simulink model "pgfm_ctrl_analysis"  (R2026b)
settings: Solver=ode23t  StopTime=param.sim.simlength  FixedStep=param.sim.tc  MaxStep=param.glb_time.tc  RelTol=1e-4
values from neighbouring files (symbols this model uses):
  param = add_template_extras(param, options)    [init_model.m]
undefined symbols (not defined in the file or in its folder): magnitude
libraries: fl_lib x99, nesl_utility x59, afe_uvw_ctrl x15, discrete_time_low_pass_filter x3, threephase_inductor_lib x3, dclink_for_two_levels x3, three_phase_pwm_modulator x3, ideal_bridges_lib x3, lithium_ion_battery x1, three_phase_voltage_with_frt_emulator_mfcn x1
(part 3 of 6)

== system pgfm_ctrl_analysis/afe_abc_inv_psm_mod2/afe/three_phase_inverter_ideal_switch_based_model ==
  gate_commands : Inport
  PS Terminator : fl_lib/Physical Signals/Sinks/PS Terminator
  PS Terminator1 : fl_lib/Physical Signals/Sinks/PS Terminator
  Simulink-PS Converter : nesl_utility/Simulink-PS Converter  PhysicalDomain=network_engine_domain  SubClassName=ps_input  LeftPortType=input  RightPortType=output  PseudoPeriodic=off  Frequencies=[]  NoiseDistribution=none  NoiseParameters=[]  Unit=V  AffineConversion=off  FilteringAndDerivatives=provide  SimscapeFilterOrder=1  InputFilterTimeConstant=0.001  UdotUserProvided=0
  Three-Phase Bridge (ideal) : ideal_bridges_lib/Three-Phase Bridge (ideal)  Vth=2.5 V  Ron=1e-3 Ohm  Goff=1e-6 1/Ohm  cap_dc=ideal_bridges.onoff.on  Cdc=2e-3 F  Vdc0=0 V  ind_ac=ideal_bridges.onoff.on  L=1e-3 H  RL=10e-3 Ohm  vdc_specify=off  vdc_priority=None  vdc=0 V  vdc_nominal_specify=off  vdc_nominal_value=1  vdc_nominal_unit=V  ic_specify=off  ic_priority=None  ic=0 A  ic_nominal_specify=off  ic_nominal_value=1  ic_nominal_unit=A  vm_a_specify=off  vm_a_priority=None  vm_a=0 V  vm_a_nominal_specify=off  vm_a_nominal_value=1  vm_a_nominal_unit=V  vm_b_specify=off  vm_b_priority=None  vm_b=0 V  vm_b_nominal_specify=off  vm_b_nominal_value=1  vm_b_nominal_unit=V  vm_c_specify=off  vm_c_priority=None  vm_c=0 V  vm_c_nominal_specify=off  vm_c_nominal_value=1  vm_c_nominal_unit=V  i_ah_specify=off  i_ah_priority=None  i_ah=0 A  i_ah_nominal_specify=off  i_ah_nominal_value=1  i_ah_nominal_unit=A  i_al_specify=off  i_al_priority=None  i_al=0 A  i_al_nominal_specify=off  i_al_nominal_value=1  i_al_nominal_unit=A  i_bh_specify=off  i_bh_priority=None  i_bh=0 A  i_bh_nominal_specify=off  i_bh_nominal_value=1  i_bh_nominal_unit=A  i_bl_specify=off  i_bl_priority=None  i_bl=0 A  i_bl_nominal_specify=off  i_bl_nominal_value=1  i_bl_nominal_unit=A  i_ch_specify=off  i_ch_priority=None  i_ch=0 A  i_ch_nominal_specify=off  i_ch_nominal_value=1  i_ch_nominal_unit=A  i_cl_specify=off  i_cl_priority=None  i_cl=0 A  i_cl_nominal_specify=off  i_cl_nominal_value=1  i_cl_nominal_unit=A  i_a_specify=off  i_a_priority=None  i_a=0 A  i_a_nominal_specify=off  i_a_nominal_value=1  i_a_nominal_unit=A  i_b_specify=off  i_b_priority=None  i_b=0 A  i_b_nominal_specify=off  i_b_nominal_value=1  i_b_nominal_unit=A  i_c_specify=off  i_c_priority=None  i_c=0 A  i_c_nominal_specify=off  i_c_nominal_value=1  i_c_nominal_unit=A
  udc(+) : PMIOPort  Side=Left
  u : PMIOPort  Port=2  Side=Right
  v : PMIOPort  Port=3  Side=Right
  udc(-) : PMIOPort  Port=4  Side=Left
  w : PMIOPort  Port=5  Side=Right
  wires:
  gate_commands/1 -> Simulink-PS Converter/1
  connections:
  PS Terminator1/LConn1 -- Three-Phase Bridge (ideal)/LConn4
  PS Terminator/LConn1 -- Three-Phase Bridge (ideal)/LConn3
  Simulink-PS Converter/RConn1 -- Three-Phase Bridge (ideal)/RConn4
  Three-Phase Bridge (ideal)/RConn1 -- u/RConn1
  Three-Phase Bridge (ideal)/LConn2 -- udc(-)/RConn1
  Three-Phase Bridge (ideal)/RConn2 -- v/RConn1
  Three-Phase Bridge (ideal)/RConn3 -- w/RConn1
  Three-Phase Bridge (ideal)/LConn1 -- udc(+)/RConn1

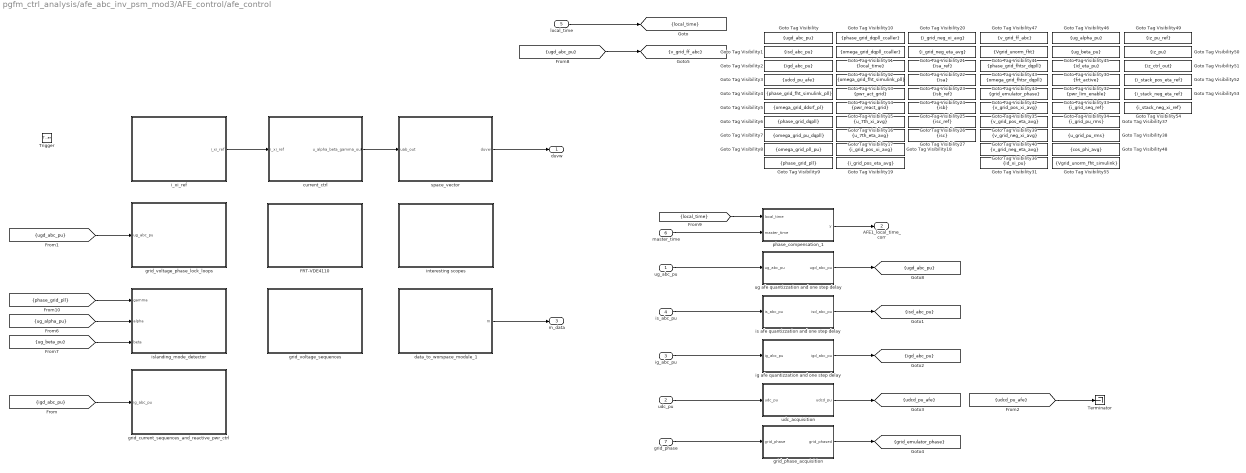
== system pgfm_ctrl_analysis/afe_abc_inv_psm_mod3/AFE_control/afe_control ==
  ug_abc_pu : Inport
  udc_pu : Inport  Port=2
  ig_abc_pu : Inport  Port=3
  is_abc_pu : Inport  Port=4
  local_time : Inport  Port=5
  master_time : Inport  Port=6
  grid_phase : Inport  Port=7
  Trigger : TriggerPort  VariantControl=(inherit)  PortDimensions=1
  FRT-VDE4110 : Subsystem
  Goto Tag Visibility : GotoTagVisibility  GotoTag=ugd_abc_pu
  Goto Tag Visibility1 : GotoTagVisibility  GotoTag=isd_abc_pu
  Goto Tag Visibility10 : GotoTagVisibility  GotoTag=phase_grid_dqpll_ccaller
  Goto Tag Visibility11 : GotoTagVisibility  GotoTag=omega_grid_dqpll_ccaller
  Goto Tag Visibility12 : GotoTagVisibility  GotoTag=local_time
  Goto Tag Visibility13 : GotoTagVisibility  GotoTag=omega_grid_fht_simulink_pll
  Goto Tag Visibility14 : GotoTagVisibility  GotoTag=pwr_act_grid
  Goto Tag Visibility15 : GotoTagVisibility  GotoTag=pwr_react_grid
  Goto Tag Visibility16 : GotoTagVisibility  GotoTag=u_7th_xi_avg
  Goto Tag Visibility17 : GotoTagVisibility  GotoTag=u_7th_eta_avg
  Goto Tag Visibility18 : GotoTagVisibility  GotoTag=i_grid_pos_xi_avg
  Goto Tag Visibility19 : GotoTagVisibility  GotoTag=i_grid_pos_eta_avg
  Goto Tag Visibility2 : GotoTagVisibility  GotoTag=igd_abc_pu
  Goto Tag Visibility20 : GotoTagVisibility  GotoTag=i_grid_neg_xi_avg
  Goto Tag Visibility21 : GotoTagVisibility  GotoTag=i_grid_neg_eta_avg
  Goto Tag Visibility22 : GotoTagVisibility  GotoTag=isa_ref
  Goto Tag Visibility23 : GotoTagVisibility  GotoTag=isa
  Goto Tag Visibility24 : GotoTagVisibility  GotoTag=isb_ref
  Goto Tag Visibility25 : GotoTagVisibility  GotoTag=isb
  Goto Tag Visibility26 : GotoTagVisibility  GotoTag=isc_ref
  Goto Tag Visibility27 : GotoTagVisibility  GotoTag=isc
  Goto Tag Visibility3 : GotoTagVisibility  GotoTag=udcd_pu_afe
  Goto Tag Visibility30 : GotoTagVisibility  GotoTag=id_eta_pu
  Goto Tag Visibility31 : GotoTagVisibility  GotoTag=id_xi_pu
  Goto Tag Visibility32 : GotoTagVisibility  GotoTag=frt_active
  Goto Tag Visibility33 : GotoTagVisibility  GotoTag=pwr_lim_enable
  Goto Tag Visibility34 : GotoTagVisibility  GotoTag=i_grid_seq_ref
  Goto Tag Visibility35 : GotoTagVisibility  GotoTag=v_grid_pos_xi_avg
  Goto Tag Visibility36 : GotoTagVisibility  GotoTag=v_grid_neg_eta_avg
  Goto Tag Visibility37 : GotoTagVisibility  GotoTag=i_grid_pu_rms
  Goto Tag Visibility38 : GotoTagVisibility  GotoTag=u_grid_pu_rms
  Goto Tag Visibility39 : GotoTagVisibility  GotoTag=v_grid_pos_eta_avg
  Goto Tag Visibility4 : GotoTagVisibility  GotoTag=phase_grid_fht_simulink_pll
  Goto Tag Visibility40 : GotoTagVisibility  GotoTag=v_grid_neg_xi_avg
  Goto Tag Visibility41 : GotoTagVisibility  GotoTag=Vgrid_unorm_fht
  Goto Tag Visibility42 : GotoTagVisibility  GotoTag=grid_emulator_phase
  Goto Tag Visibility43 : GotoTagVisibility  GotoTag=phase_grid_fhtsr_dqpll
  Goto Tag Visibility44 : GotoTagVisibility  GotoTag=omega_grid_fhtsr_dqpll
  Goto Tag Visibility45 : GotoTagVisibility  GotoTag=ug_beta_pu
  Goto Tag Visibility46 : GotoTagVisibility  GotoTag=ug_alpha_pu
  Goto Tag Visibility47 : GotoTagVisibility  GotoTag=v_grid_ff_abc
  Goto Tag Visibility48 : GotoTagVisibility  GotoTag=cos_phi_avg
  Goto Tag Visibility49 : GotoTagVisibility  GotoTag=iz_pu_ref
  Goto Tag Visibility5 : GotoTagVisibility  GotoTag=omega_grid_ddsrf_pl
  Goto Tag Visibility50 : GotoTagVisibility  GotoTag=iz_pu
  Goto Tag Visibility51 : GotoTagVisibility  GotoTag=iz_ctrl_out
  Goto Tag Visibility52 : GotoTagVisibility  GotoTag=i_stack_pos_eta_ref
  Goto Tag Visibility53 : GotoTagVisibility  GotoTag=i_stack_neg_eta_ref
  Goto Tag Visibility54 : GotoTagVisibility  GotoTag=i_stack_neg_xi_ref
  Goto Tag Visibility55 : GotoTagVisibility  GotoTag=Vgrid_unorm_fht_simulink
  Goto Tag Visibility6 : GotoTagVisibility  GotoTag=phase_grid_dqpll
  Goto Tag Visibility7 : GotoTagVisibility  GotoTag=omega_grid_pu_dqpll
  Goto Tag Visibility8 : GotoTagVisibility  GotoTag=omega_grid_pll_pu
  Goto Tag Visibility9 : GotoTagVisibility  GotoTag=phase_grid_pll
  Terminator : Terminator
  current_ctrl : Subsystem
  data_to_worspace_module_1 : Subsystem
  grid_current_sequences_and_reactive_pwr_ctrl : Subsystem
  grid_phase_acquisition : Subsystem
  grid_voltage_phase_lock_loops : Subsystem
  grid_voltage_sequences : Subsystem
  i_xi_ref : Subsystem
  ig afe quantizzation and one step delay : Subsystem
  interesting scopes : Subsystem
  is afe quantizzation and one step delay : Subsystem
  islanding_mode_detector : Subsystem
  phase_compensation_1 : Subsystem
  space_vector : Subsystem
  udc_acquisition : Subsystem
  ug afe quantizzation and one step delay : Subsystem
  duvw : Outport
  AFE1_local_time_corr : Outport  Port=2
  m_data : Outport  Port=3
  tag scope: grid_emulator_phase=scoped, igd_abc_pu=scoped, isd_abc_pu=scoped, local_time=scoped, udcd_pu_afe=scoped, ugd_abc_pu=scoped, v_grid_ff_abc=scoped
  wires:
  ug_abc_pu/1 -> ug afe quantizzation and one step delay/1(ug_abc_pu)
  space_vector/1(duvw) -> duvw/1
  is_abc_pu/1 -> is afe quantizzation and one step delay/1(is_abc_pu)
  ig_abc_pu/1 -> ig afe quantizzation and one step delay/1(ig_abc_pu)
  [ugd_abc_pu] -> grid_voltage_phase_lock_loops/1(ug_abc_pu)
  [igd_abc_pu] -> grid_current_sequences_and_reactive_pwr_ctrl/1(ig_abc_pu)
  udc_pu/1 -> udc_acquisition/1(udc_pu)
  udc_acquisition/1(udcd_pu) -> [udcd_pu_afe]
  [phase_grid_pll] -> islanding_mode_detector/1(gamma)
  [ug_alpha_pu] -> islanding_mode_detector/2(alpha)
  ug afe quantizzation and one step delay/1(ugd_abc_pu) -> [ugd_abc_pu]
  is afe quantizzation and one step delay/1(isd_abc_pu) -> [isd_abc_pu]
  ig afe quantizzation and one step delay/1(igd_abc_pu) -> [igd_abc_pu]
  [ug_beta_pu] -> islanding_mode_detector/3(beta)
  local_time/1 -> [local_time]
  master_time/1 -> phase_compensation_1/2(master_time)
  phase_compensation_1/1(y) -> AFE1_local_time_corr/1
  [local_time] -> phase_compensation_1/1(local_time)
  grid_phase/1 -> grid_phase_acquisition/1(grid_phase)
  grid_phase_acquisition/1(grid_phased) -> [grid_emulator_phase]
  [ugd_abc_pu] -> [v_grid_ff_abc]
  data_to_worspace_module_1/1(m) -> m_data/1
  [udcd_pu_afe] -> Terminator/1
  current_ctrl/1(u_alpha_beta_gamma_out) -> space_vector/1(uab_out)
  i_xi_ref/1(i_xi_ref) -> current_ctrl/1(i_xi_ref)

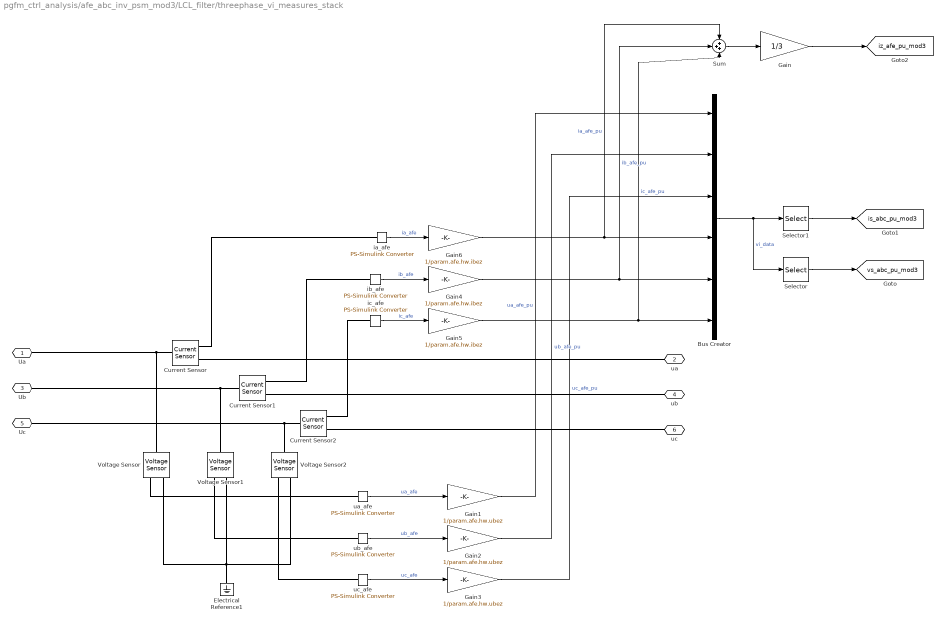
== system pgfm_ctrl_analysis/afe_abc_inv_psm_mod3/LCL_filter/threephase_vi_measures_stack ==
  Bus Creator : BusCreator  Inputs=6
  Current Sensor : fl_lib/Electrical/Electrical Sensors/Current Sensor
  Current Sensor1 : fl_lib/Electrical/Electrical Sensors/Current Sensor
  Current Sensor2 : fl_lib/Electrical/Electrical Sensors/Current Sensor
  Electrical Reference1 : fl_lib/Electrical/Electrical Elements/Electrical Reference
  Gain : Gain  Gain=1/3
  Gain1 : Gain  Gain=1/param.afe.hw.ubez
  Gain2 : Gain  Gain=1/param.afe.hw.ubez
  Gain3 : Gain  Gain=1/param.afe.hw.ubez
  Gain4 : Gain  Gain=1/param.afe.hw.ibez
  Gain5 : Gain  Gain=1/param.afe.hw.ibez
  Gain6 : Gain  Gain=1/param.afe.hw.ibez
  Selector : Selector  InputPortWidth=6  IndexOptions=Index vector (dialog)  Indices=[1 2 3]  OutputSizes=1  RuntimeRangeChecks=off
  Selector1 : Selector  InputPortWidth=6  IndexOptions=Index vector (dialog)  Indices=[4 5 6]  OutputSizes=1  RuntimeRangeChecks=off
  Sum : Sum  Inputs=+++
  Voltage Sensor : fl_lib/Electrical/Electrical Sensors/Voltage Sensor
  Voltage Sensor1 : fl_lib/Electrical/Electrical Sensors/Voltage Sensor
  Voltage Sensor2 : fl_lib/Electrical/Electrical Sensors/Voltage Sensor
  ia_afe : nesl_utility/PS-Simulink Converter  PhysicalDomain=network_engine_domain  SubClassName=ps_output  LeftPortType=input  RightPortType=output  PseudoPeriodic=off  Frequencies=[]  VectorFormat=1-D array  Unit=A  AffineConversion=off
  ib_afe : nesl_utility/PS-Simulink Converter  PhysicalDomain=network_engine_domain  SubClassName=ps_output  LeftPortType=input  RightPortType=output  PseudoPeriodic=off  Frequencies=[]  VectorFormat=1-D array  Unit=A  AffineConversion=off
  ic_afe : nesl_utility/PS-Simulink Converter  PhysicalDomain=network_engine_domain  SubClassName=ps_output  LeftPortType=input  RightPortType=output  PseudoPeriodic=off  Frequencies=[]  VectorFormat=1-D array  Unit=A  AffineConversion=off
  ua_afe : nesl_utility/PS-Simulink Converter  PhysicalDomain=network_engine_domain  SubClassName=ps_output  LeftPortType=input  RightPortType=output  PseudoPeriodic=off  Frequencies=[]  VectorFormat=1-D array  Unit=V  AffineConversion=off
  ub_afe : nesl_utility/PS-Simulink Converter  PhysicalDomain=network_engine_domain  SubClassName=ps_output  LeftPortType=input  RightPortType=output  PseudoPeriodic=off  Frequencies=[]  VectorFormat=1-D array  Unit=V  AffineConversion=off
  uc_afe : nesl_utility/PS-Simulink Converter  PhysicalDomain=network_engine_domain  SubClassName=ps_output  LeftPortType=input  RightPortType=output  PseudoPeriodic=off  Frequencies=[]  VectorFormat=1-D array  Unit=V  AffineConversion=off
  Ua : PMIOPort  Side=Left
  ua : PMIOPort  Port=2  Side=Right
  Ub : PMIOPort  Port=3  Side=Left
  ub : PMIOPort  Port=4  Side=Right
  Uc : PMIOPort  Port=5  Side=Left
  uc : PMIOPort  Port=6  Side=Right
  tag scope: is_abc_pu_mod3=global, iz_afe_pu_mod3=global, vs_abc_pu_mod3=global
  wires:
  Bus Creator/1 -> Selector/1, Selector1/1  "vi_data"
  Selector/1 -> [vs_abc_pu_mod3]
  ib_afe/1 -> Gain4/1  "ib_afe"
  ia_afe/1 -> Gain6/1  "ia_afe"
  ic_afe/1 -> Gain5/1  "ic_afe"
  ua_afe/1 -> Gain1/1  "ua_afe"
  ub_afe/1 -> Gain2/1  "ub_afe"
  uc_afe/1 -> Gain3/1  "uc_afe"
  Selector1/1 -> [is_abc_pu_mod3]
  Sum/1 -> Gain/1
  Gain/1 -> [iz_afe_pu_mod3]
  Gain1/1 -> Bus Creator/1  "ua_afe_pu"
  Gain2/1 -> Bus Creator/2  "ub_afe_pu"
  Gain3/1 -> Bus Creator/3  "uc_afe_pu"
  Gain6/1 -> Sum/1, Bus Creator/4  "ia_afe_pu"
  Gain4/1 -> Sum/2, Bus Creator/5  "ib_afe_pu"
  Gain5/1 -> Bus Creator/6, Sum/3  "ic_afe_pu"
  connections:
  Current Sensor1/LConn1 -- Ub/RConn1 -- Voltage Sensor1/LConn1
  Electrical Reference1/LConn1 -- Voltage Sensor/RConn2 -- Voltage Sensor2/RConn2 -- Voltage Sensor1/RConn2
  Voltage Sensor/RConn1 -- ua_afe/LConn1
  Current Sensor/RConn2 -- ua/RConn1
  Voltage Sensor1/RConn1 -- ub_afe/LConn1
  Voltage Sensor2/LConn1 -- Uc/RConn1 -- Current Sensor2/LConn1
  Current Sensor/LConn1 -- Ua/RConn1 -- Voltage Sensor/LConn1
  Current Sensor1/RConn2 -- ub/RConn1
  Voltage Sensor2/RConn1 -- uc_afe/LConn1
  ib_afe/LConn1 -- Current Sensor1/RConn1
  ia_afe/LConn1 -- Current Sensor/RConn1
  ic_afe/LConn1 -- Current Sensor2/RConn1
  Current Sensor2/RConn2 -- uc/RConn1

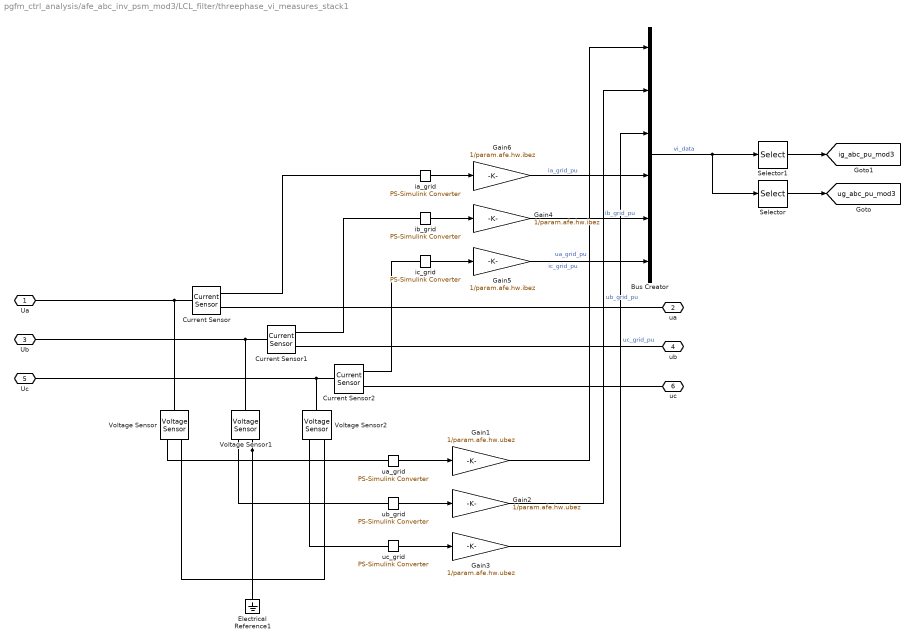
== system pgfm_ctrl_analysis/afe_abc_inv_psm_mod3/LCL_filter/threephase_vi_measures_stack1 ==
  Bus Creator : BusCreator  Inputs=6
  Current Sensor : fl_lib/Electrical/Electrical Sensors/Current Sensor
  Current Sensor1 : fl_lib/Electrical/Electrical Sensors/Current Sensor
  Current Sensor2 : fl_lib/Electrical/Electrical Sensors/Current Sensor
  Electrical Reference1 : fl_lib/Electrical/Electrical Elements/Electrical Reference
  Gain1 : Gain  Gain=1/param.afe.hw.ubez
  Gain2 : Gain  Gain=1/param.afe.hw.ubez
  Gain3 : Gain  Gain=1/param.afe.hw.ubez
  Gain4 : Gain  Gain=1/param.afe.hw.ibez
  Gain5 : Gain  Gain=1/param.afe.hw.ibez
  Gain6 : Gain  Gain=1/param.afe.hw.ibez
  Selector : Selector  InputPortWidth=6  IndexOptions=Index vector (dialog)  Indices=[1 2 3]  OutputSizes=1  RuntimeRangeChecks=off
  Selector1 : Selector  InputPortWidth=6  IndexOptions=Index vector (dialog)  Indices=[4 5 6]  OutputSizes=1  RuntimeRangeChecks=off
  Voltage Sensor : fl_lib/Electrical/Electrical Sensors/Voltage Sensor
  Voltage Sensor1 : fl_lib/Electrical/Electrical Sensors/Voltage Sensor
  Voltage Sensor2 : fl_lib/Electrical/Electrical Sensors/Voltage Sensor
  ia_grid : nesl_utility/PS-Simulink Converter  PhysicalDomain=network_engine_domain  SubClassName=ps_output  LeftPortType=input  RightPortType=output  PseudoPeriodic=off  Frequencies=[]  VectorFormat=1-D array  Unit=A  AffineConversion=off
  ib_grid : nesl_utility/PS-Simulink Converter  PhysicalDomain=network_engine_domain  SubClassName=ps_output  LeftPortType=input  RightPortType=output  PseudoPeriodic=off  Frequencies=[]  VectorFormat=1-D array  Unit=A  AffineConversion=off
  ic_grid : nesl_utility/PS-Simulink Converter  PhysicalDomain=network_engine_domain  SubClassName=ps_output  LeftPortType=input  RightPortType=output  PseudoPeriodic=off  Frequencies=[]  VectorFormat=1-D array  Unit=A  AffineConversion=off
  ua_grid : nesl_utility/PS-Simulink Converter  PhysicalDomain=network_engine_domain  SubClassName=ps_output  LeftPortType=input  RightPortType=output  PseudoPeriodic=off  Frequencies=[]  VectorFormat=1-D array  Unit=V  AffineConversion=off
  ub_grid : nesl_utility/PS-Simulink Converter  PhysicalDomain=network_engine_domain  SubClassName=ps_output  LeftPortType=input  RightPortType=output  PseudoPeriodic=off  Frequencies=[]  VectorFormat=1-D array  Unit=V  AffineConversion=off
  uc_grid : nesl_utility/PS-Simulink Converter  PhysicalDomain=network_engine_domain  SubClassName=ps_output  LeftPortType=input  RightPortType=output  PseudoPeriodic=off  Frequencies=[]  VectorFormat=1-D array  Unit=V  AffineConversion=off
  Ua : PMIOPort  Side=Left
  ua : PMIOPort  Port=2  Side=Right
  Ub : PMIOPort  Port=3  Side=Left
  ub : PMIOPort  Port=4  Side=Right
  Uc : PMIOPort  Port=5  Side=Left
  uc : PMIOPort  Port=6  Side=Right
  tag scope: ig_abc_pu_mod3=global, ug_abc_pu_mod3=global
  wires:
  Selector1/1 -> [ig_abc_pu_mod3]
  uc_grid/1 -> Gain3/1
  ub_grid/1 -> Gain2/1
  ua_grid/1 -> Gain1/1
  ic_grid/1 -> Gain5/1
  ia_grid/1 -> Gain6/1
  ib_grid/1 -> Gain4/1
  Selector/1 -> [ug_abc_pu_mod3]
  Bus Creator/1 -> Selector1/1, Selector/1  "vi_data"
  Gain1/1 -> Bus Creator/1  "ua_grid_pu"
  Gain2/1 -> Bus Creator/2  "ub_grid_pu"
  Gain3/1 -> Bus Creator/3  "uc_grid_pu"
  Gain6/1 -> Bus Creator/4  "ia_grid_pu"
  Gain4/1 -> Bus Creator/5  "ib_grid_pu"
  Gain5/1 -> Bus Creator/6  "ic_grid_pu"
  connections:
  Current Sensor2/RConn2 -- uc/RConn1
  ic_grid/LConn1 -- Current Sensor2/RConn1
  ia_grid/LConn1 -- Current Sensor/RConn1
  ib_grid/LConn1 -- Current Sensor1/RConn1
  Voltage Sensor2/RConn1 -- uc_grid/LConn1
  Current Sensor1/RConn2 -- ub/RConn1
  Voltage Sensor/LConn1 -- Current Sensor/LConn1 -- Ua/RConn1
  Current Sensor2/LConn1 -- Voltage Sensor2/LConn1 -- Uc/RConn1
  Voltage Sensor1/RConn1 -- ub_grid/LConn1
  Current Sensor/RConn2 -- ua/RConn1
  Voltage Sensor/RConn1 -- ua_grid/LConn1
  Voltage Sensor1/RConn2 -- Voltage Sensor2/RConn2 -- Voltage Sensor/RConn2 -- Electrical Reference1/LConn1
  Voltage Sensor1/LConn1 -- Current Sensor1/LConn1 -- Ub/RConn1

== system pgfm_ctrl_analysis/afe_abc_inv_psm_mod3/afe/sv_pwm ==
  duties_uvw : Inport
  Bus Selector2 : BusSelector  OutputSignals=du(k),dv(k),dw(k)
  Constant1 : Constant  Value=param.afe.behav.pwm_phase_shift_mod3
  modulator1 : Subsystem
  td2tc_1 : TransferFcn  Denominator=[param.glb_time.tc 1]
  td2tc_2 : TransferFcn  Denominator=[param.glb_time.tc 1]
  td2tc_3 : TransferFcn  Denominator=[param.glb_time.tc 1]
  gate_cmds : Outport
  wires:
  modulator1/1(gate_cmds) -> gate_cmds/1
  Constant1/1 -> modulator1/4(phase)
  Bus Selector2/1 -> td2tc_1/1  "<du(k)>"
  Bus Selector2/2 -> td2tc_2/1  "<dv(k)>"
  Bus Selector2/3 -> td2tc_3/1  "<dw(k)>"
  duties_uvw/1 -> Bus Selector2/1
  td2tc_1/1 -> modulator1/1(u)  "du(t)"
  td2tc_3/1 -> modulator1/3(w)  "dw(t)"
  td2tc_2/1 -> modulator1/2(v)  "dv(t)"

== system pgfm_ctrl_analysis/afe_abc_inv_psm_mod3/afe/three_phase_inverter_ideal_switch_based_model ==
  gate_commands : Inport
  PS Terminator : fl_lib/Physical Signals/Sinks/PS Terminator
  PS Terminator1 : fl_lib/Physical Signals/Sinks/PS Terminator
  Simulink-PS Converter : nesl_utility/Simulink-PS Converter  PhysicalDomain=network_engine_domain  SubClassName=ps_input  LeftPortType=input  RightPortType=output  PseudoPeriodic=off  Frequencies=[]  NoiseDistribution=none  NoiseParameters=[]  Unit=V  AffineConversion=off  FilteringAndDerivatives=provide  SimscapeFilterOrder=1  InputFilterTimeConstant=0.001  UdotUserProvided=0
  Three-Phase Bridge (ideal) : ideal_bridges_lib/Three-Phase Bridge (ideal)  Vth=2.5 V  Ron=1e-3 Ohm  Goff=1e-6 1/Ohm  cap_dc=ideal_bridges.onoff.on  Cdc=2e-3 F  Vdc0=0 V  ind_ac=ideal_bridges.onoff.on  L=1e-3 H  RL=10e-3 Ohm  vdc_specify=off  vdc_priority=None  vdc=0 V  vdc_nominal_specify=off  vdc_nominal_value=1  vdc_nominal_unit=V  ic_specify=off  ic_priority=None  ic=0 A  ic_nominal_specify=off  ic_nominal_value=1  ic_nominal_unit=A  vm_a_specify=off  vm_a_priority=None  vm_a=0 V  vm_a_nominal_specify=off  vm_a_nominal_value=1  vm_a_nominal_unit=V  vm_b_specify=off  vm_b_priority=None  vm_b=0 V  vm_b_nominal_specify=off  vm_b_nominal_value=1  vm_b_nominal_unit=V  vm_c_specify=off  vm_c_priority=None  vm_c=0 V  vm_c_nominal_specify=off  vm_c_nominal_value=1  vm_c_nominal_unit=V  i_ah_specify=off  i_ah_priority=None  i_ah=0 A  i_ah_nominal_specify=off  i_ah_nominal_value=1  i_ah_nominal_unit=A  i_al_specify=off  i_al_priority=None  i_al=0 A  i_al_nominal_specify=off  i_al_nominal_value=1  i_al_nominal_unit=A  i_bh_specify=off  i_bh_priority=None  i_bh=0 A  i_bh_nominal_specify=off  i_bh_nominal_value=1  i_bh_nominal_unit=A  i_bl_specify=off  i_bl_priority=None  i_bl=0 A  i_bl_nominal_specify=off  i_bl_nominal_value=1  i_bl_nominal_unit=A  i_ch_specify=off  i_ch_priority=None  i_ch=0 A  i_ch_nominal_specify=off  i_ch_nominal_value=1  i_ch_nominal_unit=A  i_cl_specify=off  i_cl_priority=None  i_cl=0 A  i_cl_nominal_specify=off  i_cl_nominal_value=1  i_cl_nominal_unit=A  i_a_specify=off  i_a_priority=None  i_a=0 A  i_a_nominal_specify=off  i_a_nominal_value=1  i_a_nominal_unit=A  i_b_specify=off  i_b_priority=None  i_b=0 A  i_b_nominal_specify=off  i_b_nominal_value=1  i_b_nominal_unit=A  i_c_specify=off  i_c_priority=None  i_c=0 A  i_c_nominal_specify=off  i_c_nominal_value=1  i_c_nominal_unit=A
  udc(+) : PMIOPort  Side=Left
  u : PMIOPort  Port=2  Side=Right
  v : PMIOPort  Port=3  Side=Right
  udc(-) : PMIOPort  Port=4  Side=Left
  w : PMIOPort  Port=5  Side=Right
  wires:
  gate_commands/1 -> Simulink-PS Converter/1
  connections:
  Three-Phase Bridge (ideal)/LConn1 -- udc(+)/RConn1
  Three-Phase Bridge (ideal)/RConn3 -- w/RConn1
  Three-Phase Bridge (ideal)/RConn2 -- v/RConn1
  Three-Phase Bridge (ideal)/LConn2 -- udc(-)/RConn1
  Three-Phase Bridge (ideal)/RConn1 -- u/RConn1
  Simulink-PS Converter/RConn1 -- Three-Phase Bridge (ideal)/RConn4
  PS Terminator/LConn1 -- Three-Phase Bridge (ideal)/LConn3
  PS Terminator1/LConn1 -- Three-Phase Bridge (ideal)/LConn4

== system pgfm_ctrl_analysis/grid/grid_emulator/3ph_Dyg_ssc ==
  C_lv_earth : fl_lib/Electrical/Electrical Elements/Capacitor  c=3*param.gnd.c_ac_phase F  r=param.gnd.r_ac_hf/3 Ohm  g=0 1/Ohm  i_specify=off  i_priority=None  i=0 A  i_nominal_specify=off  i_nominal_value=1  i_nominal_unit=A  v_specify=off  v_priority=None  v=0 V  v_nominal_specify=off  v_nominal_value=1  v_nominal_unit=V  vc_specify=off  vc_priority=High  vc=0 V  vc_nominal_specify=off  vc_nominal_value=1  vc_nominal_unit=V
  PS Terminator : fl_lib/Physical Signals/Sinks/PS Terminator
  PS Terminator1 : fl_lib/Physical Signals/Sinks/PS Terminator
  PS Terminator2 : fl_lib/Physical Signals/Sinks/PS Terminator
  R_star : fl_lib/Electrical/Electrical Elements/Resistor  R=param.gnd.r_star Ohm  i_specify=off  i_priority=None  i=0 A  i_nominal_specify=off  i_nominal_value=1  i_nominal_unit=A  v_specify=off  v_priority=None  v=0 V  v_nominal_specify=off  v_nominal_value=1  v_nominal_unit=V
  configurable_trafo : SimscapeComponentBlock  Description=Configurable transformer: one or two three-phase primaries (star or delta), secondary three-phase (star or delta, any clock number) or single-phase (turns distribution ws) on a three-limb core. Component configurable_transformer.configurable_transformer (pwr-control/library, foundation/electrical_machines/+configurable_transformer).  SourceFile=configurable_transformer.configurable_transformer  ComponentPath=configurable_transformer.configurable_transformer  ComponentVariants="[\"configurable_transformer.configurable_transformer\"]"  ComponentVariantNames="[\"configurable_transformer\"]"  ClassName=configurable_transformer  SchemaVersion=1  primaries=configurable_transformer.n_primaries.one  conn1=configurable_transformer.connection.delta  conn2=configurable_transformer.connection.star  clock2=0  secondary=configurable_transformer.secondary_winding.star  clock3=param.grid.emu.trafo.pu.clock3  ws=[1, -1, 0]  Sr=param.grid.emu.trafo.pwr_nom A*V  V1=param.grid.emu.trafo.u1_nom V  V2=400 V  V3=param.grid.emu.trafo.u2_nom V  fr=param.grid.emu.trafo.f_nom Hz  r1=param.grid.emu.trafo.pu.r1  l1=param.grid.emu.trafo.pu.l1  r2=0.005  l2=0.030  r3=param.grid.emu.trafo.pu.r3  l3=param.grid.emu.trafo.pu.l3  lm=param.grid.emu.trafo.pu.lm  lm0=param.grid.emu.trafo.pu.lm0  rfe=param.grid.emu.trafo.pu.rfe  i1a_specify=off  i1a_priority=None  i1a=0 A  i1a_nominal_specify=off  i1a_nominal_value=1  i1a_nominal_unit=A  i1b_specify=off  i1b_priority=None  i1b=0 A  i1b_nominal_specify=off  i1b_nominal_value=1  i1b_nominal_unit=A  i1c_specify=off  i1c_priority=None  i1c=0 A  i1c_nominal_specify=off  i1c_nominal_value=1  i1c_nominal_unit=A  i2a_specify=off  i2a_priority=None  i2a=0 A  i2a_nominal_specify=off  i2a_nominal_value=1  i2a_nominal_unit=A  i2b_specify=off  i2b_priority=None  i2b=0 A  i2b_nominal_specify=off  i2b_nominal_value=1  i2b_nominal_unit=A  i2c_specify=off  i2c_priority=None  i2c=0 A  i2c_nominal_specify=off  i2c_nominal_value=1  i2c_nominal_unit=A  i3a_specify=off  i3a_priority=None  i3a=0 A  i3a_nominal_specify=off  i3a_nominal_value=1  i3a_nominal_unit=A  i3b_specify=off  i3b_priority=None  i3b=0 A  i3b_nominal_specify=off  i3b_nominal_value=1  i3b_nominal_unit=A  i3c_specify=off  i3c_priority=None  i3c=0 A  i3c_nominal_specify=off  i3c_nominal_value=1  i3c_nominal_unit=A  i3_specify=off  i3_priority=None  i3=0 A  i3_nominal_specify=off  i3_nominal_value=1  i3_nominal_unit=A
      settings: CopyFcn=simscape.sscblock.internal.componentBlockCallback(gcbh,'COPY')  PreCopyFcn=simscape.sscblock.internal.componentBlockCallback(gcbh,'PRECOPY')  PreDeleteFcn=simscape.sscblock.internal.componentBlockCallback(gcbh,'PREDELETE')
      mask Type: Configurable Transformer
  earth : fl_lib/Electrical/Electrical Elements/Electrical Reference
  ua : PMIOPort  Side=Right
  ub : PMIOPort  Port=2  Side=Right
  uc : PMIOPort  Port=3  Side=Right
  Ua : PMIOPort  Port=4  Side=Left
  Ub : PMIOPort  Port=5  Side=Left
  Uc : PMIOPort  Port=6  Side=Left
  connections:
  Uc/RConn1 -- configurable_trafo/LConn3
  configurable_trafo/LConn2 -- Ub/RConn1
  configurable_trafo/RConn1 -- ua/RConn1
  configurable_trafo/LConn1 -- Ua/RConn1
  ub/RConn1 -- configurable_trafo/RConn2
  configurable_trafo/RConn3 -- uc/RConn1
  PS Terminator/LConn1 -- configurable_trafo/RConn5
  PS Terminator1/LConn1 -- configurable_trafo/RConn6
  configurable_trafo/RConn7 -- PS Terminator2/LConn1
  R_star/LConn1 -- configurable_trafo/RConn4 -- C_lv_earth/LConn1
  earth/LConn1 -- R_star/RConn1 -- C_lv_earth/RConn1

== system pgfm_ctrl_analysis/grid/grid_emulator/threephase_vi_measures ==
  Bus Creator : BusCreator  Inputs=6
  Current Sensor : fl_lib/Electrical/Electrical Sensors/Current Sensor
  Current Sensor1 : fl_lib/Electrical/Electrical Sensors/Current Sensor
  Current Sensor2 : fl_lib/Electrical/Electrical Sensors/Current Sensor
  Electrical Reference1 : fl_lib/Electrical/Electrical Elements/Electrical Reference
  Voltage Sensor : fl_lib/Electrical/Electrical Sensors/Voltage Sensor
  Voltage Sensor1 : fl_lib/Electrical/Electrical Sensors/Voltage Sensor
  Voltage Sensor2 : fl_lib/Electrical/Electrical Sensors/Voltage Sensor
  i : Selector  InputPortWidth=6  IndexOptions=Index vector (dialog)  Indices=[4 5 6]  OutputSizes=1  RuntimeRangeChecks=off
  ia_grid : nesl_utility/PS-Simulink Converter  PhysicalDomain=network_engine_domain  SubClassName=ps_output  LeftPortType=input  RightPortType=output  PseudoPeriodic=off  Frequencies=[]  VectorFormat=1-D array  Unit=A  AffineConversion=off
  ib_grid : nesl_utility/PS-Simulink Converter  PhysicalDomain=network_engine_domain  SubClassName=ps_output  LeftPortType=input  RightPortType=output  PseudoPeriodic=off  Frequencies=[]  VectorFormat=1-D array  Unit=A  AffineConversion=off
  ic_grid : nesl_utility/PS-Simulink Converter  PhysicalDomain=network_engine_domain  SubClassName=ps_output  LeftPortType=input  RightPortType=output  PseudoPeriodic=off  Frequencies=[]  VectorFormat=1-D array  Unit=A  AffineConversion=off
  u : Selector  InputPortWidth=6  IndexOptions=Index vector (dialog)  Indices=[1 2 3]  OutputSizes=1  RuntimeRangeChecks=off
  ua_grid : nesl_utility/PS-Simulink Converter  PhysicalDomain=network_engine_domain  SubClassName=ps_output  LeftPortType=input  RightPortType=output  PseudoPeriodic=off  Frequencies=[]  VectorFormat=1-D array  Unit=V  AffineConversion=off
  ub_grid : nesl_utility/PS-Simulink Converter  PhysicalDomain=network_engine_domain  SubClassName=ps_output  LeftPortType=input  RightPortType=output  PseudoPeriodic=off  Frequencies=[]  VectorFormat=1-D array  Unit=V  AffineConversion=off
  uc_grid : nesl_utility/PS-Simulink Converter  PhysicalDomain=network_engine_domain  SubClassName=ps_output  LeftPortType=input  RightPortType=output  PseudoPeriodic=off  Frequencies=[]  VectorFormat=1-D array  Unit=V  AffineConversion=off
  Ua : PMIOPort  Side=Left
  ua : PMIOPort  Port=2  Side=Right
  Ub : PMIOPort  Port=3  Side=Left
  ub : PMIOPort  Port=4  Side=Right
  Uc : PMIOPort  Port=5  Side=Left
  uc : PMIOPort  Port=6  Side=Right
  tag scope: i_abc_line=global, u_abc_line=global
  wires:
  Bus Creator/1 -> i/1, u/1  "vi_data"
  ib_grid/1 -> Bus Creator/5  "ib"
  ia_grid/1 -> Bus Creator/4  "ia"
  ic_grid/1 -> Bus Creator/6  "ic"
  ua_grid/1 -> Bus Creator/1  "ua"
  ub_grid/1 -> Bus Creator/2  "ub"
  uc_grid/1 -> Bus Creator/3  "uc"
  i/1 -> [i_abc_line]
  u/1 -> [u_abc_line]
  connections:
  Current Sensor1/LConn1 -- Ub/RConn1 -- Voltage Sensor1/LConn1
  Electrical Reference1/LConn1 -- Voltage Sensor/RConn2 -- Voltage Sensor2/RConn2 -- Voltage Sensor1/RConn2
  Voltage Sensor/RConn1 -- ua_grid/LConn1
  Current Sensor/RConn2 -- ua/RConn1
  Voltage Sensor1/RConn1 -- ub_grid/LConn1
  Voltage Sensor2/LConn1 -- Current Sensor2/LConn1 -- Uc/RConn1
  Current Sensor/LConn1 -- Ua/RConn1 -- Voltage Sensor/LConn1
  Current Sensor1/RConn2 -- ub/RConn1
  Voltage Sensor2/RConn1 -- uc_grid/LConn1
  ib_grid/LConn1 -- Current Sensor1/RConn1
  ia_grid/LConn1 -- Current Sensor/RConn1
  ic_grid/LConn1 -- Current Sensor2/RConn1
  Current Sensor2/RConn2 -- uc/RConn1

== system pgfm_ctrl_analysis/afe_abc_inv_psm_mod1/AFE_control/afe_control/FRT-VDE4110 ==
  Constant4 : Constant  Value=0
  Mux : Mux
  Mux1 : Mux  Inputs=2
  enable : Step  Time=param.frt.data.settle_time  FinalValue=param.frt.data.enable_frt_1 + param.frt.data.enable_frt_2
  frt_detection_output : Scope  NumInputPorts=3
      settings: ActiveDisplayYMinimum=-0.12499999999999997  ActiveDisplayYMaximum=1.125
  frt_vde4110 : afe_uvw_ctrl/frt_vde4110  p=param.afe.uvw
  positive_reactive_current_reference : Subsystem
  reset : Step  Time=0.025  InitialValue=1  FinalValue=0
  tag scope: frt_active=scoped, i_grid_seq_ref=scoped, pwr_lim_enable=scoped
  wires:
  frt_vde4110/2 -> [frt_active], frt_detection_output/2  "frt_active"
  frt_vde4110/3 -> [pwr_lim_enable], frt_detection_output/3  "pwr_lim_enable"
  frt_vde4110/4 -> frt_detection_output/1  "frt_state"
  reset/1 -> frt_vde4110/4  "reset"
  enable/1 -> frt_vde4110/3  "enable"
  [v_grid_neg_eta_avg] -> Mux/4
  [v_grid_neg_xi_avg] -> Mux/3
  [v_grid_pos_eta_avg] -> Mux/2
  [v_grid_pos_xi_avg] -> Mux/1
  Mux/1 -> frt_vde4110/1
  positive_reactive_current_reference/1(i_react_pos_ref) -> [i_react_pos_ref]
  Constant4/1 -> [i_react_neg_ref]
  frt_vde4110/1 -> [i_grid_seq_ref]
  [i_react_neg_ref] -> Mux1/2
  [i_react_pos_ref] -> Mux1/1
  Mux1/1 -> frt_vde4110/2

== system pgfm_ctrl_analysis/afe_abc_inv_psm_mod1/AFE_control/afe_control/current_ctrl ==
  i_xi_ref : Inport
  Mux : Mux  Inputs=3
  current_ctrl_uvw : afe_uvw_ctrl/current_ctrl_uvw  p=param.afe.uvw
  isa_ref/isa : Scope  NumInputPorts=2
      settings: ActiveDisplayYMinimum=-3.5647345146351177  ActiveDisplayYMaximum=2.2290599372806974
  u_alpha_beta_gamma_out : Outport
  wires:
  i_xi_ref/1 -> current_ctrl_uvw/1  "is_pos_xi_ref"
  [i_stack_neg_xi_ref] -> Mux/2  "is_neg_xi_ref"
  [i_stack_pos_eta_ref] -> Mux/1  "is_pos_eta_ref"
  [i_stack_neg_eta_ref] -> Mux/3  "is_neg_eta_ref"
  [phase_grid_pll] -> current_ctrl_uvw/4
  [isd_abc_pu] -> current_ctrl_uvw/3
  current_ctrl_uvw/1 -> u_alpha_beta_gamma_out/1
  current_ctrl_uvw/2 -> isa_ref/isa/1
  current_ctrl_uvw/3 -> isa_ref/isa/2
  Mux/1 -> current_ctrl_uvw/2

== system pgfm_ctrl_analysis/afe_abc_inv_psm_mod1/AFE_control/afe_control/data_to_worspace_module_1 ==
  Bus Creator : BusCreator  Inputs=5
  dq_pll : Subsystem
  inner_current_tracking : Subsystem
  pwr_meter : Subsystem
  sequences_data : Subsystem
  m : Outport
  wires:
  Bus Creator/1 -> m/1
  sequences_data/1(m_seq) -> Bus Creator/1  "sequences_data"
  pwr_meter/1(m_pwr_meter) -> Bus Creator/2  "pwr_meter"
  inner_current_tracking/1(m_inner_current_tracking) -> Bus Creator/3  "m_inner_current_tracking"
  [local_time] -> Bus Creator/5  "local_time"
  dq_pll/1(dqPLLs) -> Bus Creator/4  "dq_pll"

== system pgfm_ctrl_analysis/afe_abc_inv_psm_mod1/AFE_control/afe_control/grid_current_sequences_and_reactive_pwr_ctrl ==
  ig_abc_pu : Inport
  Abs : Abs  SaturateOnIntegerOverflow=off
  Demux : Demux  Outputs=3
  Demux1 : Demux
  Saturation : Saturate  UpperLimit=2  LowerLimit=0.1
  Terminator : Terminator
  grid_current_sequences_q_ctrl : afe_uvw_ctrl/grid_current_sequences_q_ctrl  p=param.afe.uvw
  tag scope: i_grid_neg_eta_avg=scoped, i_grid_neg_xi_avg=scoped, i_grid_pos_eta_avg=scoped, i_grid_pos_xi_avg=scoped, i_stack_neg_eta_ref=scoped, i_stack_neg_xi_ref=scoped, i_stack_pos_eta_ref=scoped
  wires:
  [phase_grid_pll] -> grid_current_sequences_q_ctrl/2
  ig_abc_pu/1 -> grid_current_sequences_q_ctrl/1
  grid_current_sequences_q_ctrl/1 -> Demux/1
  Demux/1 -> [i_stack_pos_eta_ref]
  grid_current_sequences_q_ctrl/2 -> Demux1/1
  Demux1/1 -> [i_grid_pos_xi_avg]
  Demux1/2 -> [i_grid_pos_eta_avg]
  Demux1/3 -> [i_grid_neg_xi_avg]
  Demux1/4 -> [i_grid_neg_eta_avg]
  grid_current_sequences_q_ctrl/3 -> Terminator/1
  [i_grid_seq_ref] -> grid_current_sequences_q_ctrl/4
  Saturation/1 -> grid_current_sequences_q_ctrl/3
  [omega_grid_pll_pu] -> Abs/1
  Abs/1 -> Saturation/1
  Demux/2 -> [i_stack_neg_xi_ref]
  Demux/3 -> [i_stack_neg_eta_ref]

== system pgfm_ctrl_analysis/afe_abc_inv_psm_mod1/AFE_control/afe_control/grid_phase_acquisition ==
  grid_phase : Inport
  Quantizer : Quantizer  QuantizationInterval=param.meas.adc_quantization
  Unit Delay : UnitDelay  SampleTime=-1
  Zero-Order Hold : ZeroOrderHold  SampleTime=-1
  grid_phased : Outport
  wires:
  Zero-Order Hold/1 -> Quantizer/1
  Unit Delay/1 -> grid_phased/1
  grid_phase/1 -> Zero-Order Hold/1
  Quantizer/1 -> Unit Delay/1

== system pgfm_ctrl_analysis/afe_abc_inv_psm_mod1/AFE_control/afe_control/grid_voltage_phase_lock_loops ==
  ug_abc_pu : Inport
  Bus Creator2 : BusCreator  Inputs=2
  FHT-PLL performance : Scope  NumInputPorts=2
      settings: ActiveDisplayYMinimum=-1.32501220703125  ActiveDisplayYMaximum=1.30987548828125  DataLoggingVariableName=ScopeData8
  FHT-PLL_simulink : Subsystem
  tag scope: omega_grid_pll_pu=scoped, phase_grid_pll=scoped
  wires:
  FHT-PLL_simulink/1(gamma_grid_fht_pll) -> [phase_grid_pll]
  FHT-PLL_simulink/2(omega_grid_fht_pll) -> [omega_grid_pll_pu]
  ug_abc_pu/1 -> FHT-PLL performance/1, FHT-PLL_simulink/1(ug_abc_pu)
  Bus Creator2/1 -> FHT-PLL performance/2
  [omega_grid_pll_pu] -> Bus Creator2/2  "omega_grid_fht_pll"
  [phase_grid_pll] -> Bus Creator2/1  "phase_grid_fht_pll"

== system pgfm_ctrl_analysis/afe_abc_inv_psm_mod1/AFE_control/afe_control/grid_voltage_sequences ==
  Abs : Abs  SaturateOnIntegerOverflow=off
  Demux : Demux
  Demux1 : Demux  Outputs=2
  Saturation : Saturate  UpperLimit=2  LowerLimit=0.1
  Terminator : Terminator
  grid_voltage_sequences1 : afe_uvw_ctrl/grid_voltage_sequences  p=param.afe.uvw
  tag scope: ug_alpha_pu=scoped, ug_beta_pu=scoped, v_grid_neg_eta_avg=scoped, v_grid_neg_xi_avg=scoped, v_grid_pos_eta_avg=scoped, v_grid_pos_xi_avg=scoped
  wires:
  [ugd_abc_pu] -> grid_voltage_sequences1/1
  [phase_grid_pll] -> grid_voltage_sequences1/2
  Abs/1 -> Saturation/1
  [omega_grid_pll_pu] -> Abs/1
  Saturation/1 -> grid_voltage_sequences1/3
  grid_voltage_sequences1/1 -> Demux/1
  Demux/4 -> [v_grid_neg_eta_avg]
  Demux/3 -> [v_grid_neg_xi_avg]
  Demux/2 -> [v_grid_pos_eta_avg]
  Demux/1 -> [v_grid_pos_xi_avg]
  grid_voltage_sequences1/3 -> Demux1/1
  Demux1/1 -> [ug_alpha_pu]
  Demux1/2 -> [ug_beta_pu]
  grid_voltage_sequences1/2 -> Terminator/1

== system pgfm_ctrl_analysis/afe_abc_inv_psm_mod1/AFE_control/afe_control/i_xi_ref ==
  Constant1 : Constant  Value=param.afe.ref.ixi_ref_mod1
  Constant2 : Constant  Value=0
  Delay : Delay  DelayLength=floor(0.25/param.glb_time.ts_afe)
  Switch : Switch  Criteria=u2 > Threshold  SaturateOnIntegerOverflow=off  InputSameDT=off
  Switch1 : Switch  Criteria=u2 > Threshold  SaturateOnIntegerOverflow=off  InputSameDT=off
  Variant Source : VariantSource  VariantControls={false, true}
  discrete-time-low-pass-filter : discrete_time_low_pass_filter/discrete-time-low-pass-filter  tau=0.125  ts=param.glb_time.ts_afe
  i_xi_ref : Outport
  wires:
  Constant1/1 -> Switch/3  "i_xi_ref"
  Constant2/1 -> Switch/1
  [pwr_lim_enable] -> Switch/2
  [pwr_lim_enable] -> Delay/1
  Switch/1 -> discrete-time-low-pass-filter/1, Variant Source/2, Switch1/3
  Delay/1 -> Switch1/2
  discrete-time-low-pass-filter/1 -> Switch1/1
  Switch1/1 -> Variant Source/1
  Variant Source/1 -> i_xi_ref/1

== system pgfm_ctrl_analysis/afe_abc_inv_psm_mod1/AFE_control/afe_control/ig afe quantizzation and one step delay ==
  ig_abc_pu : Inport
  Demux1 : Demux  Outputs=3
  Mux1 : Mux  Inputs=3
  ig afe quantizzation and one step delay : Subsystem
  igd_abc_pu : Outport
  wires:
  Demux1/1 -> ig afe quantizzation and one step delay/1(ig_u_pu)
  Demux1/2 -> ig afe quantizzation and one step delay/2(ig_v_pu)
  ig_abc_pu/1 -> Demux1/1
  Mux1/1 -> igd_abc_pu/1
  Demux1/3 -> ig afe quantizzation and one step delay/3(ig_w_pu)
  ig afe quantizzation and one step delay/2(igd_v_pu) -> Mux1/2
  ig afe quantizzation and one step delay/1(igd_u_pu) -> Mux1/1
  ig afe quantizzation and one step delay/3(igd_w_pu) -> Mux1/3

== system pgfm_ctrl_analysis/afe_abc_inv_psm_mod1/AFE_control/afe_control/interesting scopes ==
  current_sequences_mod1 : Scope  NumInputPorts=4
      settings: ActiveDisplayYMinimum=-0.97178065031766891  ActiveDisplayYMaximum=1.9392475411295891  DataLoggingVariableName=ScopeData2
  i_grid_seq_ref : Scope
      settings: ActiveDisplayYMinimum=-1.1499999999999995  ActiveDisplayYMaximum=0.34999999999999981
  voltage_sequences_mod1 : Scope  NumInputPorts=4
      settings: ActiveDisplayYMinimum=-1.2405151816982258  ActiveDisplayYMaximum=1.2605257614333911
  wires:
  [v_grid_neg_eta_avg] -> voltage_sequences_mod1/4  "u_grid_neg_eta"
  [i_grid_neg_xi_avg] -> current_sequences_mod1/3  "i_grid_neg_xi"
  [v_grid_pos_eta_avg] -> voltage_sequences_mod1/2  "u_grid_pos_eta"
  [v_grid_neg_xi_avg] -> voltage_sequences_mod1/3  "u_grid_neg_xi"
  [i_grid_pos_xi_avg] -> current_sequences_mod1/1  "i_grid_pos_xi"
  [i_grid_neg_eta_avg] -> current_sequences_mod1/4  "i_grid_neg_eta"
  [v_grid_pos_xi_avg] -> voltage_sequences_mod1/1  "u_grid_pos_xi"
  [i_grid_pos_eta_avg] -> current_sequences_mod1/2  "i_grid_pos_eta"
  [i_grid_seq_ref] -> i_grid_seq_ref/1  "i_grid_seq_ref"

== system pgfm_ctrl_analysis/afe_abc_inv_psm_mod1/AFE_control/afe_control/is afe quantizzation and one step delay ==
  is_abc_pu : Inport
  Demux : Demux  Outputs=3
  Mux : Mux  Inputs=3
  is afe quantizzation and one step delay : Subsystem
  isd_abc_pu : Outport
  wires:
  is afe quantizzation and one step delay/2(isd_v_pu) -> Mux/2
  is_abc_pu/1 -> Demux/1
  is afe quantizzation and one step delay/3(isd_w_pu) -> Mux/3
  is afe quantizzation and one step delay/1(isd_u_pu) -> Mux/1
  Demux/1 -> is afe quantizzation and one step delay/1(is_u_pu)
  Mux/1 -> isd_abc_pu/1
  Demux/3 -> is afe quantizzation and one step delay/3(is_w_pu)
  Demux/2 -> is afe quantizzation and one step delay/2(is_v_pu)

== system pgfm_ctrl_analysis/afe_abc_inv_psm_mod1/AFE_control/afe_control/islanding_mode_detector ==
  gamma : Inport
  alpha : Inport  Port=2
  beta : Inport  Port=3
  Constant : Constant
  Mux : Mux  Inputs=2
  island_detection : Scope  NumInputPorts=3
      settings: ActiveDisplayYMinimum=-13.028939727220205  ActiveDisplayYMaximum=117.26045754498188  DataLoggingVariableName=ScopeData10
  islanding_detector : afe_uvw_ctrl/islanding_detector  p=param.afe.uvw
  wires:
  Mux/1 -> islanding_detector/1
  alpha/1 -> Mux/1  "u_grid_alpha"
  beta/1 -> Mux/2  "u_grid_beta"
  gamma/1 -> islanding_detector/2  "gamma_grid"
  [omega_grid_pll_pu] -> islanding_detector/3
  Constant/1 -> islanding_detector/4
  islanding_detector/1 -> island_detection/1
  islanding_detector/2 -> island_detection/2
  islanding_detector/3 -> island_detection/3

== system pgfm_ctrl_analysis/afe_abc_inv_psm_mod1/AFE_control/afe_control/phase_compensation_1 ==
  local_time : Inport
  master_time : Inport  Port=2
  Zero-Order Hold : ZeroOrderHold  SampleTime=-1
  Zero-Order Hold1 : ZeroOrderHold  SampleTime=-1
  alignment_eval_afe1 : Subsystem
  y : Outport
  wires:
  local_time/1 -> Zero-Order Hold/1
  master_time/1 -> Zero-Order Hold1/1
  alignment_eval_afe1/1(dp) -> y/1
  Zero-Order Hold/1 -> alignment_eval_afe1/1(local_time)
  Zero-Order Hold1/1 -> alignment_eval_afe1/2(master_time)

== system pgfm_ctrl_analysis/afe_abc_inv_psm_mod1/AFE_control/afe_control/space_vector ==
  uab_out : Inport
  Bus Creator : BusCreator  Inputs=3
  Bus Selector : BusSelector  OutputSignals=da,db,dc
  C Caller : CCaller  FunctionName=sv_pwm_cm_process_simulink  PortSpecificationStruct="%)30     .    B H   8    (     @         %    \"     8    !     0         %  0 \"0    $    _    07)G3F%M90  4&]R=$YA;64 4V-O<&4     26YD97@     5'EP90      4VEZ90      27-';&]B86P   X    P    !@    @    $          4    (     0    ,    !         !   P!O=70 #@   #     &    \"     0         !0    @    !     P    $         $  # &]U=  .    .     8    (    !          %    \"     $    &     0         0   ...(+3252 chars)"
  Constant : Constant  Value=param.glb_time.ts_afe
  Constant1 : Constant
  Data Type Conversion1 : DataTypeConversion  OutDataTypeStr=double  SaturateOnIntegerOverflow=off  RndMeth=Floor
  Data Type Conversion{4,15..16,18} (4 alike) : DataTypeConversion  OutDataTypeStr=single  SaturateOnIntegerOverflow=off  RndMeth=Floor
  Data Type Conversion17 : DataTypeConversion  OutDataTypeStr=uint32  SaturateOnIntegerOverflow=off  RndMeth=Floor
  Data Type Conversion2 : DataTypeConversion  OutDataTypeStr=double  SaturateOnIntegerOverflow=off  RndMeth=Floor
  Data Type Conversion3 : DataTypeConversion  OutDataTypeStr=double  SaturateOnIntegerOverflow=off  RndMeth=Floor
  Demux : Demux  Outputs=3
  Gain1 : Gain  Gain=sqrt(3)/2
  Gain2 : Gain  Gain=sqrt(3)/2
  Gain3 : Gain  Gain=param.afe.ref.u_cm_comp_mod1
  duvw : Outport
  wires:
  Data Type Conversion15/1 -> C Caller/2
  Bus Selector/2 -> Data Type Conversion2/1  "<db>"
  Data Type Conversion18/1 -> C Caller/1
  C Caller/1 -> Bus Selector/1
  Bus Creator/1 -> duvw/1
  Data Type Conversion1/1 -> Bus Creator/1  "du(k)"
  Demux/2 -> Gain2/1
  Bus Selector/3 -> Data Type Conversion3/1  "<dc>"
  Demux/1 -> Gain1/1
  Data Type Conversion2/1 -> Bus Creator/2  "dv(k)"
  Gain2/1 -> Data Type Conversion15/1
  Bus Selector/1 -> Data Type Conversion1/1  "<da>"
  Gain1/1 -> Data Type Conversion18/1
  Data Type Conversion3/1 -> Bus Creator/3  "dw(k)"
  Constant/1 -> Data Type Conversion16/1
  uab_out/1 -> Demux/1
  Constant1/1 -> Data Type Conversion17/1
  Data Type Conversion16/1 -> C Caller/4
  Data Type Conversion17/1 -> C Caller/5
  Demux/3 -> Gain3/1
  Gain3/1 -> Data Type Conversion4/1
  Data Type Conversion4/1 -> C Caller/3

== system pgfm_ctrl_analysis/afe_abc_inv_psm_mod1/AFE_control/afe_control/udc_acquisition ==
  udc_pu : Inport
  Quantizer : Quantizer  QuantizationInterval=param.meas.adc_quantization
  Unit Delay : UnitDelay  SampleTime=-1
  Zero-Order Hold : ZeroOrderHold  SampleTime=-1
  udcd_pu : Outport
  wires:
  Quantizer/1 -> Unit Delay/1
  udc_pu/1 -> Zero-Order Hold/1
  Unit Delay/1 -> udcd_pu/1
  Zero-Order Hold/1 -> Quantizer/1

== system pgfm_ctrl_analysis/afe_abc_inv_psm_mod1/AFE_control/afe_control/ug afe quantizzation and one step delay ==
  ug_abc_pu : Inport
  Demux : Demux  Outputs=3
  Mux : Mux  Inputs=3
  ug afe quantizzation and one step delay : Subsystem
  ugd_abc_pu : Outport
  wires:
  ug afe quantizzation and one step delay/2(ugd_v_pu) -> Mux/2
  Demux/2 -> ug afe quantizzation and one step delay/2(ug_v_pu)
  Demux/3 -> ug afe quantizzation and one step delay/3(ug_w_pu)
  ug afe quantizzation and one step delay/1(ugd_u_pu) -> Mux/1
  Demux/1 -> ug afe quantizzation and one step delay/1(ug_u_pu)
  ug_abc_pu/1 -> Demux/1
  ug afe quantizzation and one step delay/3(ugd_w_pu) -> Mux/3
  Mux/1 -> ugd_abc_pu/1

== system pgfm_ctrl_analysis/afe_abc_inv_psm_mod1/afe/sv_pwm/modulator1 ==
  u : Inport
  v : Inport  Port=2
  w : Inport  Port=3
  phase : Inport  Port=4
  Bus Creator : BusCreator  Inputs=3
  Three phase two level PWM generator with global TRGO : three_phase_pwm_modulator/Three phase two level PWM generator with global TRGO  f=param.glb_time.fPWM_AFE  m_up=0.98  m_low=0.02  dead_time=param.glb_time.dead_time_AFE  pos_cmd_gate=15  neg_cmd_gate=-10  polarity=1  tc=param.glb_time.tc  double_sampling=1
      link override gate commands/Bus Selector: OutputSignals=du(t)
      link override gate commands/Bus Selector1: OutputSignals=dv(t)
      link override gate commands/Bus Selector2: OutputSignals=dw(t)
  gate_cmds : Outport
  tag scope: TRGO_afe_module_1=global
  wires:
  [time_afe_module_1] -> Three phase two level PWM generator with global TRGO/1
  Bus Creator/1 -> Three phase two level PWM generator with global TRGO/3
  Three phase two level PWM generator with global TRGO/1 -> [TRGO_afe_module_1]
  u/1 -> Bus Creator/1
  v/1 -> Bus Creator/2
  w/1 -> Bus Creator/3
  phase/1 -> Three phase two level PWM generator with global TRGO/2
  Three phase two level PWM generator with global TRGO/2 -> gate_cmds/1
